simulink model "RoadsterJump"  (R2025b)
settings: Solver=ode1  StartTime=0.0  StopTime=8  FixedStep=1e-3  RelTol=1e-3
undefined symbols (not defined in the file): plan, rtl, tBurn, xBurn
Description:
  | Jump over five vehicles. Logged signals: x, y, theta, vy, mode, F_lift, F_att, P_tank, T_tank, m_air, low, clearance. Modes: 0 roll, 1 boost, 2 coast, 3 landing burn, 4 landed.
settings Model: Creator=kichuiyer  LastModifiedBy=kichuiyer
settings DataIOCC: SaveOutput=off

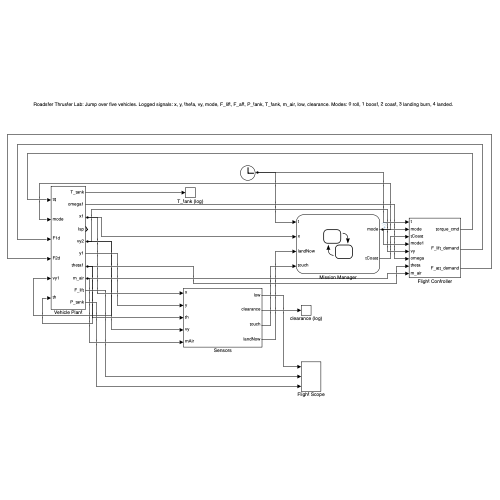
[thumbnail: Simulink's stored preview of the top-level diagram]
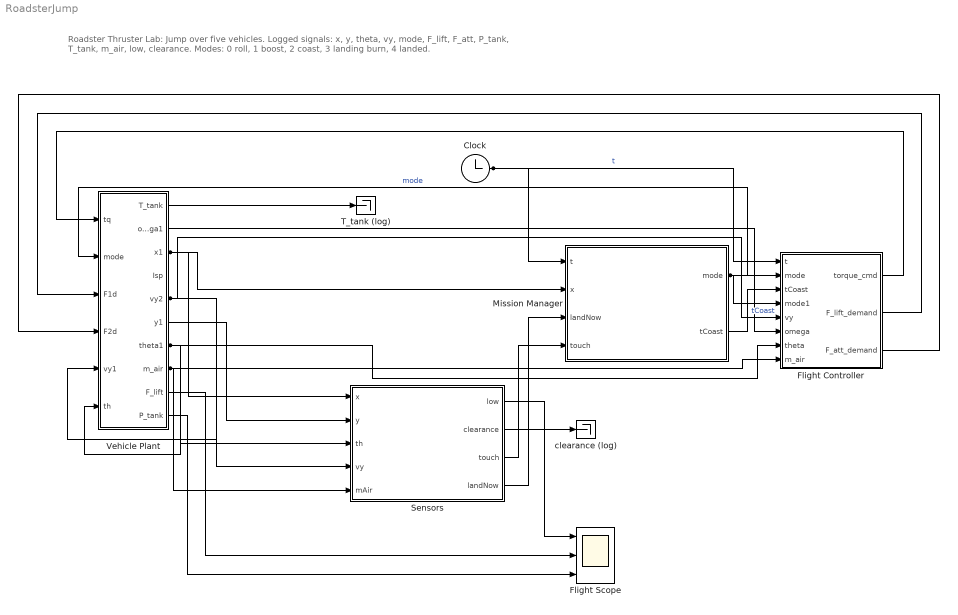
== system RoadsterJump ==
  note: Roadster Thruster Lab: Jump over five vehicles. Logged signals: x, y, theta, vy, mode, F_lift, F_att, P_tank, T_tank, m_air, low, clearance. Modes: 0 roll, 1 boost, 2 coast, 3 landing burn, 4 landed.
  Clock : Clock
  Flight Controller : Subsystem
  Flight Scope : Scope  NumInputPorts=3
  Mission Manager : Stateflow chart  TreatAsAtomicUnit=on
  Sensors : Subsystem
  T_tank (log) : Terminator
  Vehicle Plant : Subsystem
  clearance (log) : Terminator
  wires:
  Flight Controller/3(F_att_demand) -> Vehicle Plant/4(F2d)
  Flight Controller/2(F_lift_demand) -> Vehicle Plant/3(F1d)
  Flight Controller/1(torque_cmd) -> Vehicle Plant/1(tq)
  Sensors/4(landNow) -> Mission Manager/3(landNow)
  Sensors/3(touch) -> Mission Manager/4(touch)
  Vehicle Plant/8(m_air) -> Sensors/5(mAir), Flight Controller/8(m_air)
  Clock/1 -> Mission Manager/1(t), Flight Controller/1(t)  "t"
  Vehicle Plant/7(theta1) -> Sensors/3(th), Vehicle Plant/6(th), Flight Controller/7(theta)
  Mission Manager/2(tCoast) -> Flight Controller/3(tCoast)  "tCoast"
  Vehicle Plant/5(vy2) -> Sensors/4(vy), Vehicle Plant/5(vy1), Flight Controller/5(vy)
  Vehicle Plant/10(P_tank) -> Flight Scope/3
  Vehicle Plant/3(x1) -> Sensors/1(x), Mission Manager/2(x)
  Mission Manager/1(mode) -> Flight Controller/2(mode), Vehicle Plant/2(mode), Flight Controller/4(mode1)  "mode"
  Vehicle Plant/9(F_lift) -> Flight Scope/2
  Sensors/2(clearance) -> clearance (log)/1
  Vehicle Plant/2(omega1) -> Flight Controller/6(omega)
  Vehicle Plant/6(y1) -> Sensors/2(y)
  Sensors/1(low) -> Flight Scope/1
  Vehicle Plant/1(T_tank) -> T_tank (log)/1

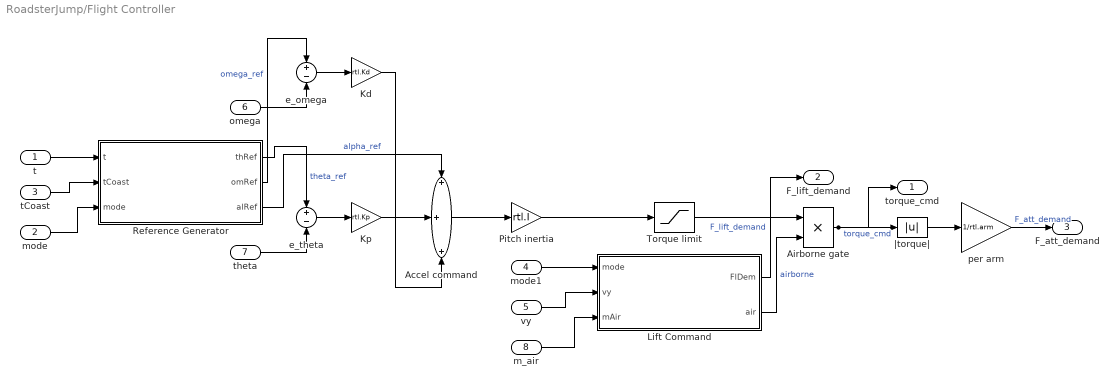
== system RoadsterJump/Flight Controller ==
  t : Inport
  mode : Inport  Port=2
  tCoast : Inport  Port=3
  mode1 : Inport  Port=4
  vy : Inport  Port=5
  omega : Inport  Port=6
  theta : Inport  Port=7
  m_air : Inport  Port=8
  Accel command : Sum  Inputs=+++
  Airborne gate : Product
  Kd : Gain  Gain=rtl.Kd
  Kp : Gain  Gain=rtl.Kp
  Lift Command : MATLAB Function  TreatAsAtomicUnit=on
  Pitch inertia : Gain  Gain=rtl.I
  Reference Generator : MATLAB Function  TreatAsAtomicUnit=on
  Torque limit : Saturate  UpperLimit=rtl.Tmax  LowerLimit=-rtl.Tmax
  e_omega : Sum  Inputs=+-
  e_theta : Sum  Inputs=+-
  per arm : Gain  Gain=1/rtl.arm
  |torque| : Abs  SaturateOnIntegerOverflow=off
  torque_cmd : Outport
  F_lift_demand : Outport  Port=2
  F_att_demand : Outport  Port=3
  wires:
  |torque|/1 -> per arm/1
  m_air/1 -> Lift Command/3(mAir)
  Lift Command/2(air) -> Airborne gate/2  "airborne"
  vy/1 -> Lift Command/2(vy)
  mode1/1 -> Lift Command/1(mode)
  Lift Command/1(FlDem) -> F_lift_demand/1  "F_lift_demand"
  Accel command/1 -> Pitch inertia/1
  Torque limit/1 -> Airborne gate/1
  Kp/1 -> Accel command/2
  e_theta/1 -> Kp/1
  Kd/1 -> Accel command/3
  Pitch inertia/1 -> Torque limit/1
  theta/1 -> e_theta/2
  per arm/1 -> F_att_demand/1  "F_att_demand"
  Reference Generator/2(omRef) -> e_omega/1  "omega_ref"
  e_omega/1 -> Kd/1
  Reference Generator/3(alRef) -> Accel command/1  "alpha_ref"
  Reference Generator/1(thRef) -> e_theta/1  "theta_ref"
  mode/1 -> Reference Generator/3(mode)
  tCoast/1 -> Reference Generator/2(tCoast)
  Airborne gate/1 -> torque_cmd/1, |torque|/1  "torque_cmd"
  omega/1 -> e_omega/2
  t/1 -> Reference Generator/1(t)

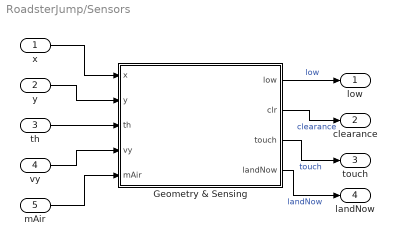
== system RoadsterJump/Sensors ==
  x : Inport
  y : Inport  Port=2
  th : Inport  Port=3
  vy : Inport  Port=4
  mAir : Inport  Port=5
  Geometry & Sensing : MATLAB Function  TreatAsAtomicUnit=on
  low : Outport
  clearance : Outport  Port=2
  touch : Outport  Port=3
  landNow : Outport  Port=4
  wires:
  Geometry & Sensing/4(landNow) -> landNow/1  "landNow"
  Geometry & Sensing/3(touch) -> touch/1  "touch"
  mAir/1 -> Geometry & Sensing/5(mAir)
  y/1 -> Geometry & Sensing/2(y)
  vy/1 -> Geometry & Sensing/4(vy)
  Geometry & Sensing/1(low) -> low/1  "low"
  th/1 -> Geometry & Sensing/3(th)
  Geometry & Sensing/2(clr) -> clearance/1  "clearance"
  x/1 -> Geometry & Sensing/1(x)

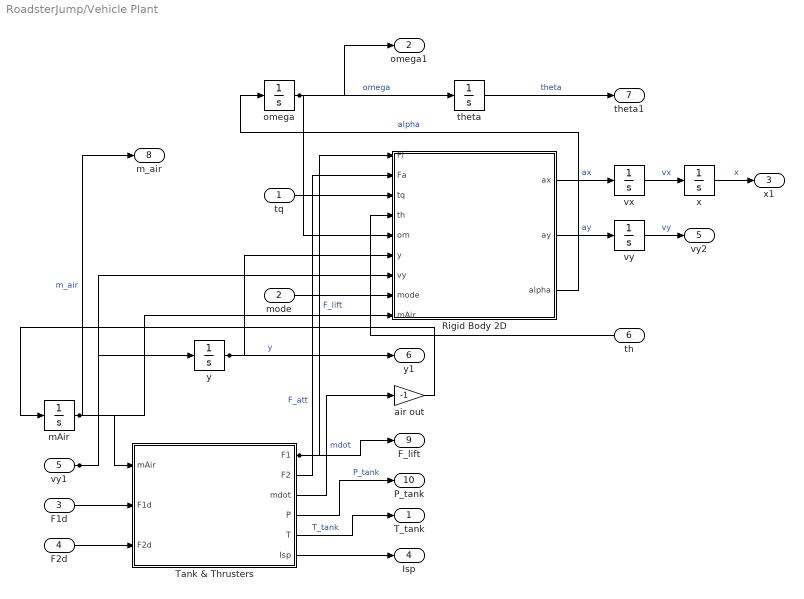
== system RoadsterJump/Vehicle Plant ==
  tq : Inport
  mode : Inport  Port=2
  F1d : Inport  Port=3
  F2d : Inport  Port=4
  vy1 : Inport  Port=5
  th : Inport  Port=6
  Rigid Body 2D : MATLAB Function  TreatAsAtomicUnit=on
  Tank & Thrusters : MATLAB Function  TreatAsAtomicUnit=on
  air out : Gain  Gain=-1
  mAir : Integrator  InitialCondition=rtl.m0  LimitOutput=on  LowerSaturationLimit=0
  omega : Integrator
  theta : Integrator
  vx : Integrator  InitialCondition=rtl.v0
  vy : Integrator
  x : Integrator  InitialCondition=plan.xStart
  y : Integrator  InitialCondition=rtl.cg
  T_tank : Outport
  omega1 : Outport  Port=2
  x1 : Outport  Port=3
  Isp : Outport  Port=4
  vy2 : Outport  Port=5
  y1 : Outport  Port=6
  theta1 : Outport  Port=7
  m_air : Outport  Port=8
  F_lift : Outport  Port=9
  P_tank : Outport  Port=10
  wires:
  x/1 -> x1/1  "x"
  vy/1 -> vy2/1  "vy"
  vx/1 -> x/1  "vx"
  th/1 -> Rigid Body 2D/4(th)
  Rigid Body 2D/2(ay) -> vy/1  "ay"
  theta/1 -> theta1/1  "theta"
  Rigid Body 2D/1(ax) -> vx/1  "ax"
  Tank & Thrusters/4(P) -> P_tank/1  "P_tank"
  Tank & Thrusters/3(mdot) -> air out/1  "mdot"
  y/1 -> y1/1, Rigid Body 2D/6(y)  "y"
  Tank & Thrusters/6(Isp) -> Isp/1
  mode/1 -> Rigid Body 2D/8(mode)
  tq/1 -> Rigid Body 2D/3(tq)
  Tank & Thrusters/2(F2) -> Rigid Body 2D/2(Fa)  "F_att"
  air out/1 -> mAir/1
  vy1/1 -> y/1, Rigid Body 2D/7(vy)
  F1d/1 -> Tank & Thrusters/2(F1d)
  Tank & Thrusters/1(F1) -> F_lift/1, Rigid Body 2D/1(Fl)  "F_lift"
  Rigid Body 2D/3(alpha) -> omega/1  "alpha"
  F2d/1 -> Tank & Thrusters/3(F2d)
  mAir/1 -> m_air/1, Tank & Thrusters/1(mAir), Rigid Body 2D/9(mAir)  "m_air"
  Tank & Thrusters/5(T) -> T_tank/1  "T_tank"
  omega/1 -> theta/1, omega1/1, Rigid Body 2D/5(om)  "omega"

== matlab function RoadsterJump/Flight Controller/Reference Generator ==
  data: t input; thRef output; tCoast input; mode input; omRef output; alRef output; rtl parameter
function [thRef, omRef, alRef] = reference(t, tCoast, mode, rtl)
%#codegen
% Pitch reference: hold level, or a minimum-jerk 360 degree flip after the burn.
thRef = 0; omRef = 0; alRef = 0;
if rtl.spin > 0 && mode >= 2 && tCoast > 0
    D = rtl.Dspin;
    u = min(1, max(0, (t - tCoast)/D));
    thRef = 2*pi*(10*u^3 - 15*u^4 + 6*u^5);
    if u < 1
        omRef = 2*pi*(30*u^2 - 60*u^3 + 30*u^4)/D;
        alRef = 2*pi*(60*u - 180*u^2 + 120*u^3)/D^2;
    end
end

== matlab function RoadsterJump/Sensors/Geometry & Sensing ==
  data: x input; low output; y input; th input; vy input; mAir input; clr output; touch output; landNow output; rtl parameter
function [low, clr, touch, landNow] = geometry(x, y, th, vy, mAir, rtl)
%#codegen
% Lowest point of the car body, clearance over the vehicle row, and the
% landing-burn trigger (stopping distance at the available deceleration).
px = [linspace(-2.2, 2.2, 9), linspace(-2.2, 2.2, 9), -2.2, 2.2, -1.35, 1.35];
py = [-0.42*ones(1,9), 0.58*ones(1,9), 0.08, -0.15, -0.55, -0.55];
c = cos(th); s = sin(th);
low = 1e9; clr = 99;
for i = 1:numel(px)
    wx = x + px(i)*c - py(i)*s;
    wy = y + px(i)*s + py(i)*c;
    low = min(low, wy);
    for k = 1:size(rtl.obs, 1)
        if wx >= rtl.obs(k,1) && wx <= rtl.obs(k,2)
            clr = min(clr, wy - rtl.obs(k,3));
        end
    end
end
touch = double(low <= 0 && vy < 0);
r  = max(mAir, 1e-6)/rtl.m0;
pc = min(rtl.Preg, rtl.P0*r^rtl.gam);
an = rtl.FliftMax*(pc/rtl.Preg)/(rtl.dry + mAir) - rtl.g0;
e  = th - 2*pi*round(th/(2*pi));
landNow = 0;
if vy < 0 && an > 0 && abs(e) < 0.25 && low <= vy^2/(2*an) + 0.3
    landNow = 1;
end

== stateflow chart RoadsterJump/Mission Manager ==
  settings: updateMethod=DISCRETE  sampleTime=1e-3
  state ROLL
    entry: mode = 0;
  state BOOST
    entry: mode = 1; tb = t;
  state COAST
    entry: mode = 2; tCoast = t;
  state LANDED
    entry: mode = 4;
  state LANDING_BURN
    entry: mode = 3;
  (default) -> ROLL
  ROLL -> BOOST : [x >= xBurn]
  BOOST -> COAST [order 1] : [t >= tb + tBurn]
  BOOST -> LANDED [order 2] : [touch > 0.5 && t > tb + 0.05]
  COAST -> LANDED [order 2] : [touch > 0.5]
  COAST -> LANDING_BURN [order 1] : [landNow > 0.5]
  LANDING_BURN -> LANDED : [touch > 0.5]
  data: t input; x input; landNow input; touch input; mode output double; tCoast output double; tb local double; xBurn parameter; tBurn parameter

== matlab function RoadsterJump/Flight Controller/Lift Command ==
  data: mode input; FlDem output; vy input; mAir input; air output; rtl parameter
function [FlDem, air] = lift_command(mode, vy, mAir, rtl)
%#codegen
% Boost: full lift. Landing burn: track a 1 m/s descent. Otherwise off.
m = rtl.dry + mAir;
FlDem = 0;
if mode == 1
    FlDem = rtl.FliftMax;
elseif mode == 3
    FlDem = min(rtl.FliftMax, max(0, m*(rtl.g0 + 8*(-1.0 - vy))));
end
air = double(mode >= 1 && mode <= 3);

== matlab function RoadsterJump/Vehicle Plant/Tank & Thrusters ==
  data: mAir input; F1 output; F1d input; F2d input; F2 output; mdot output; P output; T output; Isp output; rtl parameter
function [F1, F2, mdot, P, T, Isp] = tank_thrusters(mAir, F1d, F2d, rtl)
%#codegen
% Cold-gas tank with adiabatic blowdown feeding regulated, choked nozzles.
r   = max(mAir, 1e-6) / rtl.m0;
P   = rtl.P0 * r^rtl.gam;              % isentropic: gas left behind expands
T   = rtl.T0 * r^(rtl.gam - 1);        % ...and cools
pc  = min(rtl.Preg, P);                % regulator caps the nozzle feed
Cf  = rtl.CFm + (pc*rtl.PR - rtl.Pa)/pc*rtl.eps;
Isp = Cf * sqrt(rtl.R*T/rtl.gam) / rtl.CK / rtl.g0;
k   = pc / rtl.Preg;
if pc < 15e5, k = 0; end               % too little pressure to run
F1  = max(F1d, 0) * k;
F2  = max(F2d, 0) * k;
mdot = (F1 + F2) / (Isp * rtl.g0);     % rocket equation: mdot = F/(Isp g0)

== matlab function RoadsterJump/Vehicle Plant/Rigid Body 2D ==
  data: Fl input; ax output; Fa input; tq input; th input; om input; y input; vy input; mode input; mAir input; ay output; alpha output; rtl parameter
function [ax, ay, alpha] = rigid_body(Fl, Fa, tq, th, om, y, vy, mode, mAir, rtl)
%#codegen
% Planar rigid body. Lift acts along the body normal; attitude jets give torque.
% After landing, a stiff spring-damper stands in for tyres and suspension.
m = rtl.dry + mAir;
ax = 0; ay = 0; alpha = 0;
if mode >= 1 && mode <= 3
    ax = -sin(th)*Fl/m;
    ay =  cos(th)*Fl/m - rtl.g0;
    alpha = sign(tq)*Fa*rtl.arm/rtl.I;
elseif mode == 4
    thR = 2*pi*round(th/(2*pi));
    ay = 900*(rtl.cg - y) - 60*vy;
    alpha = 900*(thR - th) - 60*om;
end
